simulink model "test_RNN_harness"  (R2025b)
settings: Solver=FixedStepAuto  StartTime=0.0  StopTime=5  FixedStep=Ts  RelTol=1e-3
values from neighbouring files (symbols this model uses):
  Ts = 0.05    [test_RNN.m]
settings Model: Creator=Max  LastModifiedBy=nicol
settings SolverCC: AlgebraicLoopSolver=TrustRegion
settings DebuggingCC: UnconnectedInputMsg=warning  UnconnectedOutputMsg=warning  UnconnectedLineMsg=warning
settings ModelReferenceCC: EnableRefExpFcnMdlSchedulingChecks=on
settings RTWCC: GPUComputeCapability=3.5

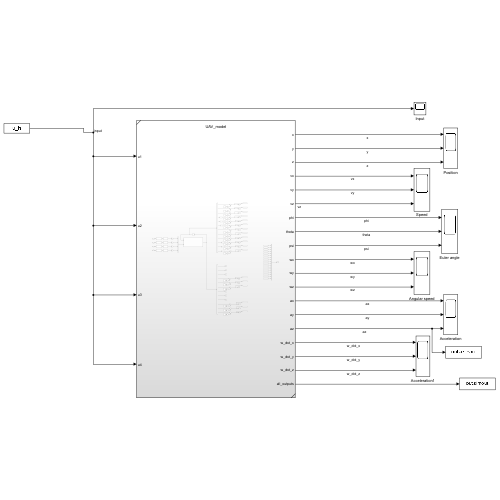
[thumbnail: Simulink's stored preview of the top-level diagram]
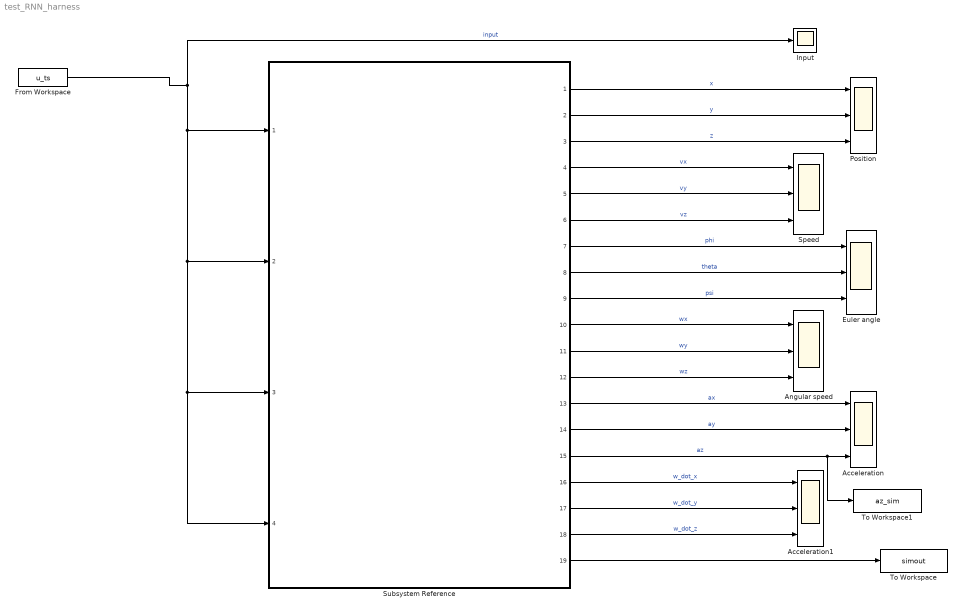
== system test_RNN_harness ==
  Acceleration : Scope  NumInputPorts=3
      settings: ActiveDisplayYMinimum=-35.48317  ActiveDisplayYMaximum=15.8515
  Acceleration1 : Scope  NumInputPorts=3
      settings: ActiveDisplayYMinimum=-1052.98102  ActiveDisplayYMaximum=116.99789  DataLoggingVariableName=ScopeData2
  Angular speed : Scope  NumInputPorts=3
      settings: ActiveDisplayYMinimum=-0.45167  ActiveDisplayYMaximum=0.49611  DataLoggingVariableName=ScopeData3
  Euler angle : Scope  NumInputPorts=3
      settings: ActiveDisplayYMinimum=-1695.66598  ActiveDisplayYMaximum=1344.64163  DataLoggingVariableName=ScopeData4
  From Workspace : FromWorkspace  VariableName=u_ts  SampleTime=Ts  Interpolate=off  OutputAfterFinalValue=Holding final value
  Input : Scope
      settings: ActiveDisplayYMinimum=-1.21244  ActiveDisplayYMaximum=1.20985  DataLoggingVariableName=ScopeData5
  Position : Scope  NumInputPorts=3
      settings: ActiveDisplayYMinimum=-1052.98102  ActiveDisplayYMaximum=116.99789  DataLoggingVariableName=ScopeData6
  Speed : Scope  NumInputPorts=3
      settings: ActiveDisplayYMinimum=-1193.81123  ActiveDisplayYMaximum=133.09449
  Subsystem Reference : Subsystem  ReferencedSubsystem=UAV_model
  To Workspace : ToWorkspace  VariableName=simout  SaveFormat=Structure With Time  SampleTime=Ts
  To Workspace1 : ToWorkspace  VariableName=az_sim  SampleTime=Ts
  wires:
  Subsystem Reference/18 -> Acceleration1/3  "w_dot_z"
  Subsystem Reference/12 -> Angular speed/3  "wz"
  Subsystem Reference/17 -> Acceleration1/2  "w_dot_y"
  Subsystem Reference/9 -> Euler angle/3  "psi"
  Subsystem Reference/8 -> Euler angle/2  "theta"
  Subsystem Reference/14 -> Acceleration/2  "ay"
  Subsystem Reference/10 -> Angular speed/1  "wx"
  Subsystem Reference/2 -> Position/2  "y"
  Subsystem Reference/13 -> Acceleration/1  "ax"
  Subsystem Reference/15 -> To Workspace1/1, Acceleration/3  "az"
  Subsystem Reference/16 -> Acceleration1/1  "w_dot_x"
  Subsystem Reference/7 -> Euler angle/1  "phi"
  Subsystem Reference/19 -> To Workspace/1
  Subsystem Reference/1 -> Position/1  "x"
  Subsystem Reference/6 -> Speed/3  "vz"
  Subsystem Reference/4 -> Speed/1  "vx"
  From Workspace/1 -> Subsystem Reference/1, Subsystem Reference/4, Subsystem Reference/3, Subsystem Reference/2, Input/1  "input"
  Subsystem Reference/3 -> Position/3  "z"
  Subsystem Reference/5 -> Speed/2  "vy"
  Subsystem Reference/11 -> Angular speed/2  "wy"
